simulink model "Transformer_Operating_Model_backup_before_callback_fix"  (R2025b)
settings: Solver=ode23t  StartTime=0.0  StopTime=t_stop  MaxStep=t_step_max  RelTol=1e-3
PreLoadFcn:
  | params_transformer;
InitFcn:
  | params_transformer;
undefined symbols (not defined in the file or in its folder): dT_double_age, dTheta_hr, I_LV_rated, k21, P0, P_load_min, P_tot_r, Pk, R_th_h, S_rated, theta_amb_C, theta_ref_age, x_oil, y_wdg
libraries: fl_lib x16, nesl_utility x10, ee_lib x4
settings Model: Creator=Silas Asare  LastModifiedBy=Silas Asare

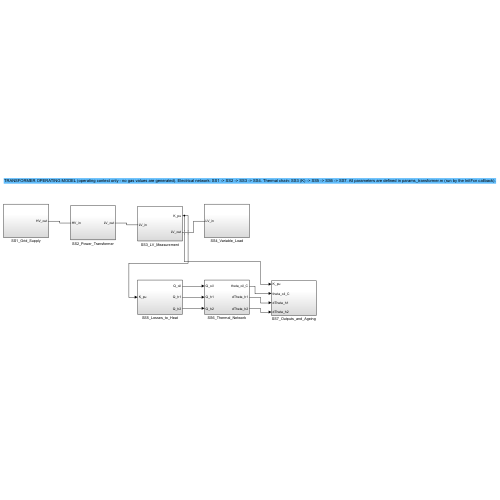
[thumbnail: Simulink's stored preview of the top-level diagram]
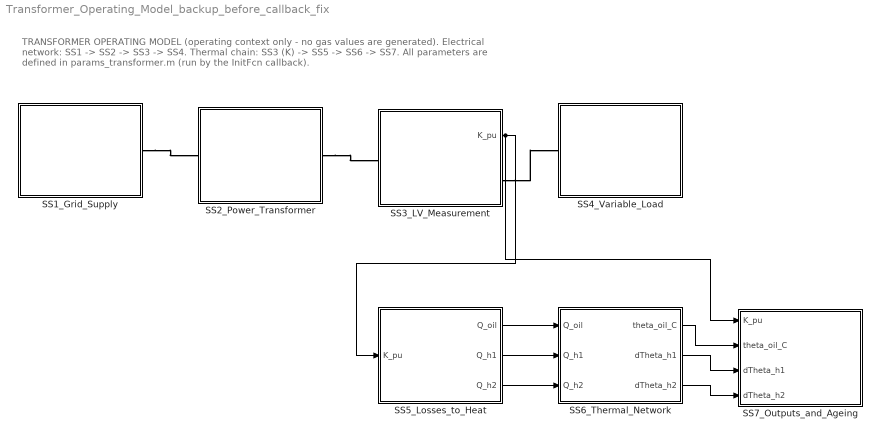
== system Transformer_Operating_Model_backup_before_callback_fix ==
  note: TRANSFORMER OPERATING MODEL (operating context only - no gas values are generated). Electrical network: SS1 -> SS2 -> SS3 -> SS4. Thermal chain: SS3 (K) -> SS5 -> SS6 -> SS7. All parameters are defined in params_transformer.m (run by the InitFcn callback).
  SS1_Grid_Supply : Subsystem
  SS2_Power_Transformer : Subsystem
  SS3_LV_Measurement : Subsystem
  SS4_Variable_Load : Subsystem
  SS5_Losses_to_Heat : Subsystem
  SS6_Thermal_Network : Subsystem
  SS7_Outputs_and_Ageing : Subsystem
  wires:
  SS3_LV_Measurement/1(K_pu) -> SS5_Losses_to_Heat/1(K_pu), SS7_Outputs_and_Ageing/1(K_pu)
  SS5_Losses_to_Heat/1(Q_oil) -> SS6_Thermal_Network/1(Q_oil)
  SS6_Thermal_Network/1(theta_oil_C) -> SS7_Outputs_and_Ageing/2(theta_oil_C)
  SS5_Losses_to_Heat/2(Q_h1) -> SS6_Thermal_Network/2(Q_h1)
  SS6_Thermal_Network/2(dTheta_h1) -> SS7_Outputs_and_Ageing/3(dTheta_h1)
  SS5_Losses_to_Heat/3(Q_h2) -> SS6_Thermal_Network/3(Q_h2)
  SS6_Thermal_Network/3(dTheta_h2) -> SS7_Outputs_and_Ageing/4(dTheta_h2)
  connections:
  SS1_Grid_Supply/RConn1 -- SS2_Power_Transformer/LConn1
  SS2_Power_Transformer/RConn1 -- SS3_LV_Measurement/LConn1
  SS3_LV_Measurement/RConn1 -- SS4_Variable_Load/LConn1

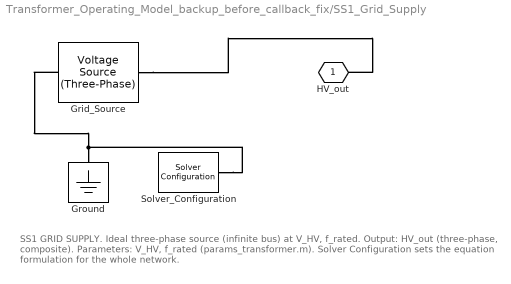
== system Transformer_Operating_Model_backup_before_callback_fix/SS1_Grid_Supply ==
  note: SS1 GRID SUPPLY. Ideal three-phase source (infinite bus) at V_HV, f_rated. Output: HV_out (three-phase, composite). Parameters: V_HV, f_rated (params_transformer.m). Solver Configuration sets the equation formulation for the whole network.
  Grid_Source : ee_lib/Sources/Voltage Source (Three-Phase)  vline_rms=V_HV V  shift=phase_shift_deg deg  freq=f_rated Hz  impedance_option=0  SShortCircuit=1e6 A*V  XR=15  R=0.01 Ohm  L=3.97e-4 H  harmonic_option=0  harmonic_orders=[5, 7, 11, 13]  harmonic_ratios=[.1, .1, .1, .1]  G_parasitic=0 1/Ohm  I_specify=off  I_priority=None  I=[0, 0, 0] A  I_nominal_specify=off  I_nominal_value=1  I_nominal_unit=A
  Ground : fl_lib/Electrical/Electrical Elements/Electrical Reference
  Solver_Configuration : nesl_utility/Solver Configuration  PhysicalDomain=network_engine_domain  SubClassName=solver  LeftPortType=input  RightPortType=generic  Tones=[]  Harmonics=[]  SimulateNoise=off  Profile=off  UseLocalSampling=off  EnableSwitchedLinearOptims=on  FrequencyDomain=off  UseCCode=off  RelTol=0.001  AbsTol=0.001  MinStep=1e-09  ToWorkspace=off  RevertToSquareIcSolve=off  NumHomotopyIterations=100  PhasorMode=off  PhasorModeNumHarmonics=1  ConsistencySolver=NEWTON_XTOL_AFTER_FTOL  IndexReductionMethod=DerivativeReplacement  DoDC=off  ResidualTolerance=1e-09  ConsistencyTolSource=GLOBAL  ConsistencyAbsTol=0.001  ConsistencyRelTol=0.001  ConsistencyTolFactor=0.001  UseLocalSolver=off  LocalSolverChoice=NE_BACKWARD_EULER_ADVANCER  ResolveIndetEquations=on  FunctionEvalNumThread=1  LocalSolverSampleTime=0.001  DoFixedCost=off  MaxNonlinIter=3  MaxModeIter=2  ComputeImpulses=off  ImpulseIterations=2  LinearAlgebra=auto  LinearAlgebraNumThread=0  EquationFormulation=NE_FREQUENCY_TIME_EF  DelaysMemoryBudget=1024  AutomaticFiltering=on  FilteringTimeConstant=0.001  PartitionStorageMethod=AS_NEEDED  PartitionMemoryBudget=1024  PartitionMethod=ROBUST  MultibodyUseLocalSolver=off  MultibodyLocalSolverChoice=ODE1  MultibodyLocalSolverSampleTime=0.001
  HV_out : PMIOPort  Side=Right
  connections:
  Ground/LConn1 -- Grid_Source/LConn1 -- Solver_Configuration/RConn1
  Grid_Source/RConn1 -- HV_out/RConn1

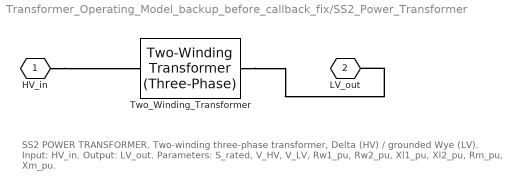
== system Transformer_Operating_Model_backup_before_callback_fix/SS2_Power_Transformer ==
  note: SS2 POWER TRANSFORMER. Two-winding three-phase transformer, Delta (HV) / grounded Wye (LV). Input: HV_in. Output: LV_out. Parameters: S_rated, V_HV, V_LV, Rw1_pu, Rw2_pu, Xl1_pu, Xl2_pu, Rm_pu, Xm_pu.
  Two_Winding_Transformer : ee_lib/Passive/Transformers/Two-Winding Transformer (Three-Phase)  SRated=S_rated V*A  FRated=f_rated Hz  Winding1Connection=ee.enum.windingconnection.delta1  VRated1=V_HV V  Winding2Connection=ee.enum.windingconnection.Yg  VRated2=V_LV V  CoreType=ee.enum.coretype.threelimb  pu_Rw1=Rw1_pu  pu_Rw2=Rw2_pu  leakage_reactance_option=ee.enum.transformer_leakage.include  pu_Xl1=Xl1_pu  pu_Xl2=Xl2_pu  magnetizing_resistance_option=ee.enum.transformer_magnetizingResistance.include  pu_Rm=Rm_pu  magnetizing_reactance_option=ee.enum.transformer_magnetizingReactance.include  saturation_option=ee.enum.transformer_saturation.exclude  pu_Xm=Xm_pu  current_data=[0, .002, 1, 2]  magnetic_flux_data=[0, 1.2, 1.5, 1.51]  pu_X0=0.5  i1_specify=off  i1_priority=None  i1=[0, 0, 0] A  i1_nominal_specify=off  i1_nominal_value=1  i1_nominal_unit=A  i2_specify=off  i2_priority=None  i2=[0, 0, 0] A  i2_nominal_specify=off  i2_nominal_value=1  i2_nominal_unit=A  phi_specify=off  phi_priority=None  phi=[0, 0, 0]  phi_nominal_specify=off  phi_nominal_value=1  phi_nominal_unit=1  power_dissipated_specify=off  power_dissipated_priority=None  power_dissipated=0 W  power_dissipated_nominal_specify=off  power_dissipated_nominal_value=1  power_dissipated_nominal_unit=W
      settings: InternalSimscapePortConfiguration="{\"Bottom\":[],\"Left\":[{\"id\":\"N1\",\"label\":\"~1\",\"type\":\"foundation.electrical.three_phase\"}],\"Right\":[{\"id\":\"N2\",\"label\":\"~2\",\"type\":\"foundation.electrical.three_phase\"}],\"Top\":[]}"
  HV_in : PMIOPort  Side=Left
  LV_out : PMIOPort  Port=2  Side=Right
  connections:
  HV_in/RConn1 -- Two_Winding_Transformer/LConn1
  Two_Winding_Transformer/RConn1 -- LV_out/RConn1

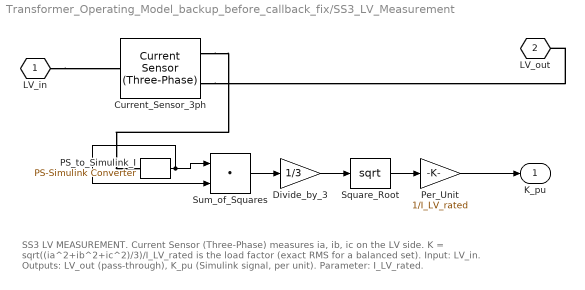
== system Transformer_Operating_Model_backup_before_callback_fix/SS3_LV_Measurement ==
  note: SS3 LV MEASUREMENT. Current Sensor (Three-Phase) measures ia, ib, ic on the LV side. K = sqrt((ia^2+ib^2+ic^2)/3)/I_LV_rated is the load factor (exact RMS for a balanced set). Input: LV_in. Outputs: LV_out (pass-through), K_pu (Simulink signal, per unit). Parameter: I_LV_rated.
  Current_Sensor_3ph : ee_lib/Sensors & Transducers/Current Sensor (Three-Phase)
  Divide_by_3 : Gain  Gain=1/3
  PS_to_Simulink_I : nesl_utility/PS-Simulink Converter  PhysicalDomain=network_engine_domain  SubClassName=ps_output  LeftPortType=input  RightPortType=output  PseudoPeriodic=off  Frequencies=[]  VectorFormat=inherit  Unit=A  AffineConversion=off
  Per_Unit : Gain  Gain=1/I_LV_rated
  Square_Root : Math  Operator=sqrt
  Sum_of_Squares : DotProduct  OutDataTypeStr=Inherit: Inherit via internal rule
  LV_in : PMIOPort  Side=Left
  LV_out : PMIOPort  Port=2  Side=Right
  K_pu : Outport
  wires:
  PS_to_Simulink_I/1 -> Sum_of_Squares/1, Sum_of_Squares/2
  Sum_of_Squares/1 -> Divide_by_3/1
  Divide_by_3/1 -> Square_Root/1
  Square_Root/1 -> Per_Unit/1
  Per_Unit/1 -> K_pu/1
  connections:
  LV_in/RConn1 -- Current_Sensor_3ph/LConn1
  Current_Sensor_3ph/RConn2 -- LV_out/RConn1
  Current_Sensor_3ph/RConn1 -- PS_to_Simulink_I/LConn1

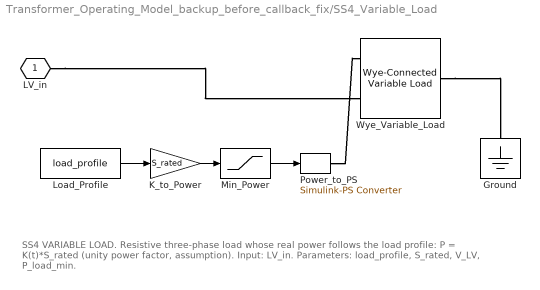
== system Transformer_Operating_Model_backup_before_callback_fix/SS4_Variable_Load ==
  note: SS4 VARIABLE LOAD. Resistive three-phase load whose real power follows the load profile: P = K(t)*S_rated (unity power factor, assumption). Input: LV_in. Parameters: load_profile, S_rated, V_LV, P_load_min.
  Ground : fl_lib/Electrical/Electrical Elements/Electrical Reference
  K_to_Power : Gain  Gain=S_rated
  Load_Profile : FromWorkspace  VariableName=load_profile  OutputAfterFinalValue=Holding final value
  Min_Power : Saturate  UpperLimit=inf  LowerLimit=P_load_min
  Power_to_PS : nesl_utility/Simulink-PS Converter  PhysicalDomain=network_engine_domain  SubClassName=ps_input  LeftPortType=input  RightPortType=output  PseudoPeriodic=off  Frequencies=[]  NoiseDistribution=none  NoiseParameters=[]  Unit=W  AffineConversion=off  FilteringAndDerivatives=provide  SimscapeFilterOrder=1  InputFilterTimeConstant=0.001  UdotUserProvided=0
  Wye_Variable_Load : ee_lib/Passive/RLC Assemblies/Wye-Connected Variable Load  VRated=V_LV V  Pmin=P_load_min W
      settings: InternalSimscapePortConfiguration="{\"Bottom\":[],\"Left\":[{\"id\":\"P\",\"label\":\"P\",\"type\":\"input\"},{\"id\":\"N\",\"label\":\"~\",\"type\":\"foundation.electrical.three_phase\"}],\"Right\":[{\"id\":\"n\",\"label\":\"n\",\"type\":\"foundation.electrical.electrical\"}],\"Top\":[]}"
  LV_in : PMIOPort  Side=Left
  wires:
  Load_Profile/1 -> K_to_Power/1
  K_to_Power/1 -> Min_Power/1
  Min_Power/1 -> Power_to_PS/1
  connections:
  LV_in/RConn1 -- Wye_Variable_Load/LConn2
  Wye_Variable_Load/RConn1 -- Ground/LConn1
  Power_to_PS/RConn1 -- Wye_Variable_Load/LConn1

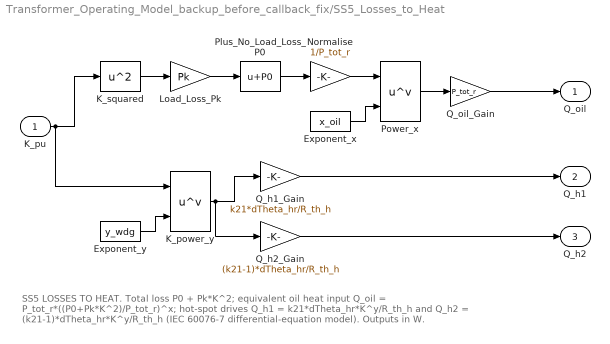
== system Transformer_Operating_Model_backup_before_callback_fix/SS5_Losses_to_Heat ==
  note: SS5 LOSSES TO HEAT. Total loss P0 + Pk*K^2; equivalent oil heat input Q_oil = P_tot_r*((P0+Pk*K^2)/P_tot_r)^x; hot-spot drives Q_h1 = k21*dTheta_hr*K^y/R_th_h and Q_h2 = (k21-1)*dTheta_hr*K^y/R_th_h (IEC 60076-7 differential-equation model). Outputs in W.
  K_pu : Inport
  Exponent_x : Constant  Value=x_oil
  Exponent_y : Constant  Value=y_wdg
  K_power_y : Math  Operator=pow
  K_squared : Math  Operator=square
  Load_Loss_Pk : Gain  Gain=Pk
  Normalise : Gain  Gain=1/P_tot_r
  Plus_No_Load_Loss_P0 : Bias  Bias=P0  SaturateOnIntegerOverflow=off
  Power_x : Math  Operator=pow
  Q_h1_Gain : Gain  Gain=k21*dTheta_hr/R_th_h
  Q_h2_Gain : Gain  Gain=(k21-1)*dTheta_hr/R_th_h
  Q_oil_Gain : Gain  Gain=P_tot_r
  Q_oil : Outport
  Q_h1 : Outport  Port=2
  Q_h2 : Outport  Port=3
  wires:
  K_pu/1 -> K_squared/1, K_power_y/1
  K_squared/1 -> Load_Loss_Pk/1
  Load_Loss_Pk/1 -> Plus_No_Load_Loss_P0/1
  Plus_No_Load_Loss_P0/1 -> Normalise/1
  Normalise/1 -> Power_x/1
  Exponent_x/1 -> Power_x/2
  Power_x/1 -> Q_oil_Gain/1
  Q_oil_Gain/1 -> Q_oil/1
  Exponent_y/1 -> K_power_y/2
  K_power_y/1 -> Q_h1_Gain/1, Q_h2_Gain/1
  Q_h1_Gain/1 -> Q_h1/1
  Q_h2_Gain/1 -> Q_h2/1

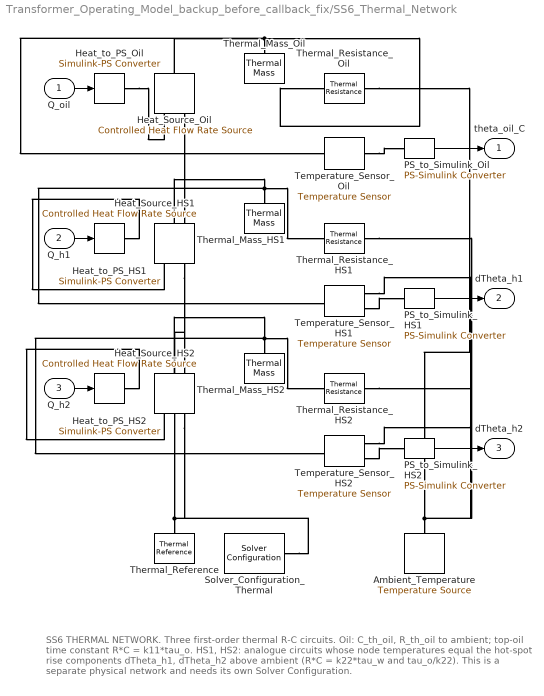
== system Transformer_Operating_Model_backup_before_callback_fix/SS6_Thermal_Network ==
  note: SS6 THERMAL NETWORK. Three first-order thermal R-C circuits. Oil: C_th_oil, R_th_oil to ambient; top-oil time constant R*C = k11*tau_o. HS1, HS2: analogue circuits whose node temperatures equal the hot-spot rise components dTheta_h1, dTheta_h2 above ambient (R*C = k22*tau_w and tau_o/k22). This is a separate physical network and needs its own Solver Configuration.
  Q_oil : Inport
  Q_h1 : Inport  Port=2
  Q_h2 : Inport  Port=3
  Ambient_Temperature : fl_lib/Thermal/Thermal Sources/Temperature Source  temperature=theta_amb_C + 273.15 K
  Heat_Source_HS1 : fl_lib/Thermal/Thermal Sources/Controlled Heat Flow Rate Source
  Heat_Source_HS2 : fl_lib/Thermal/Thermal Sources/Controlled Heat Flow Rate Source
  Heat_Source_Oil : fl_lib/Thermal/Thermal Sources/Controlled Heat Flow Rate Source
  Heat_to_PS_HS1 : nesl_utility/Simulink-PS Converter  PhysicalDomain=network_engine_domain  SubClassName=ps_input  LeftPortType=input  RightPortType=output  PseudoPeriodic=off  Frequencies=[]  NoiseDistribution=none  NoiseParameters=[]  Unit=W  AffineConversion=off  FilteringAndDerivatives=provide  SimscapeFilterOrder=1  InputFilterTimeConstant=0.001  UdotUserProvided=0
  Heat_to_PS_HS2 : nesl_utility/Simulink-PS Converter  PhysicalDomain=network_engine_domain  SubClassName=ps_input  LeftPortType=input  RightPortType=output  PseudoPeriodic=off  Frequencies=[]  NoiseDistribution=none  NoiseParameters=[]  Unit=W  AffineConversion=off  FilteringAndDerivatives=provide  SimscapeFilterOrder=1  InputFilterTimeConstant=0.001  UdotUserProvided=0
  Heat_to_PS_Oil : nesl_utility/Simulink-PS Converter  PhysicalDomain=network_engine_domain  SubClassName=ps_input  LeftPortType=input  RightPortType=output  PseudoPeriodic=off  Frequencies=[]  NoiseDistribution=none  NoiseParameters=[]  Unit=W  AffineConversion=off  FilteringAndDerivatives=provide  SimscapeFilterOrder=1  InputFilterTimeConstant=0.001  UdotUserProvided=0
  PS_to_Simulink_HS1 : nesl_utility/PS-Simulink Converter  PhysicalDomain=network_engine_domain  SubClassName=ps_output  LeftPortType=input  RightPortType=output  PseudoPeriodic=off  Frequencies=[]  VectorFormat=inherit  Unit=K  AffineConversion=off
  PS_to_Simulink_HS2 : nesl_utility/PS-Simulink Converter  PhysicalDomain=network_engine_domain  SubClassName=ps_output  LeftPortType=input  RightPortType=output  PseudoPeriodic=off  Frequencies=[]  VectorFormat=inherit  Unit=K  AffineConversion=off
  PS_to_Simulink_Oil : nesl_utility/PS-Simulink Converter  PhysicalDomain=network_engine_domain  SubClassName=ps_output  LeftPortType=input  RightPortType=output  PseudoPeriodic=off  Frequencies=[]  VectorFormat=inherit  Unit=degC  AffineConversion=on
  Solver_Configuration_Thermal : nesl_utility/Solver Configuration  PhysicalDomain=network_engine_domain  SubClassName=solver  LeftPortType=input  RightPortType=generic  Tones=[]  Harmonics=[]  SimulateNoise=off  Profile=off  UseLocalSampling=off  EnableSwitchedLinearOptims=on  FrequencyDomain=off  UseCCode=off  RelTol=0.001  AbsTol=0.001  MinStep=1e-09  ToWorkspace=off  RevertToSquareIcSolve=off  NumHomotopyIterations=100  PhasorMode=off  PhasorModeNumHarmonics=1  ConsistencySolver=NEWTON_XTOL_AFTER_FTOL  IndexReductionMethod=DerivativeReplacement  DoDC=off  ResidualTolerance=1e-09  ConsistencyTolSource=GLOBAL  ConsistencyAbsTol=0.001  ConsistencyRelTol=0.001  ConsistencyTolFactor=0.001  UseLocalSolver=off  LocalSolverChoice=NE_BACKWARD_EULER_ADVANCER  ResolveIndetEquations=on  FunctionEvalNumThread=1  LocalSolverSampleTime=0.001  DoFixedCost=off  MaxNonlinIter=3  MaxModeIter=2  ComputeImpulses=off  ImpulseIterations=2  LinearAlgebra=auto  LinearAlgebraNumThread=0  EquationFormulation=NE_TIME_EF  DelaysMemoryBudget=1024  AutomaticFiltering=on  FilteringTimeConstant=0.001  PartitionStorageMethod=AS_NEEDED  PartitionMemoryBudget=1024  PartitionMethod=ROBUST  MultibodyUseLocalSolver=off  MultibodyLocalSolverChoice=ODE1  MultibodyLocalSolverSampleTime=0.001
  Temperature_Sensor_HS1 : fl_lib/Thermal/Thermal Sensors/Temperature Sensor  temperature_measure=foundation.enum.MeasurementReference.difference
  Temperature_Sensor_HS2 : fl_lib/Thermal/Thermal Sensors/Temperature Sensor  temperature_measure=foundation.enum.MeasurementReference.difference
  Temperature_Sensor_Oil : fl_lib/Thermal/Thermal Sensors/Temperature Sensor  temperature_measure=foundation.enum.MeasurementReference.absolute
      settings: InternalSimscapePortConfiguration="{\"Bottom\":[],\"Left\":[{\"id\":\"A\",\"label\":\"A\",\"type\":\"foundation.thermal.thermal\"}],\"Right\":[{\"id\":\"T\",\"label\":\"T\",\"type\":\"output\"}],\"Top\":[]}"
  Thermal_Mass_HS1 : fl_lib/Thermal/Thermal Elements/Thermal Mass  mass_type=foundation.enum.constant_variable.constant  mass=C_th_h1 kg  sp_heat=cp_unit J/(kg*K)  mass_min=1e-6 kg  num_ports=foundation.enum.numPorts2.one  m_specify=off  m_priority=High  m=1 kg  m_nominal_specify=off  m_nominal_value=1  m_nominal_unit=kg  T_specify=on  T_priority=High  T=theta_amb_C + 273.15 K  T_nominal_specify=off  T_nominal_value=1  T_nominal_unit=K  Q_specify=off  Q_priority=None  Q=0 W  Q_nominal_specify=off  Q_nominal_value=1  Q_nominal_unit=W
  Thermal_Mass_HS2 : fl_lib/Thermal/Thermal Elements/Thermal Mass  mass_type=foundation.enum.constant_variable.constant  mass=C_th_h2 kg  sp_heat=cp_unit J/(kg*K)  mass_min=1e-6 kg  num_ports=foundation.enum.numPorts2.one  m_specify=off  m_priority=High  m=1 kg  m_nominal_specify=off  m_nominal_value=1  m_nominal_unit=kg  T_specify=on  T_priority=High  T=theta_amb_C + 273.15 K  T_nominal_specify=off  T_nominal_value=1  T_nominal_unit=K  Q_specify=off  Q_priority=None  Q=0 W  Q_nominal_specify=off  Q_nominal_value=1  Q_nominal_unit=W
  Thermal_Mass_Oil : fl_lib/Thermal/Thermal Elements/Thermal Mass  mass_type=foundation.enum.constant_variable.constant  mass=C_th_oil kg  sp_heat=cp_unit J/(kg*K)  mass_min=1e-6 kg  num_ports=foundation.enum.numPorts2.one  m_specify=off  m_priority=High  m=1 kg  m_nominal_specify=off  m_nominal_value=1  m_nominal_unit=kg  T_specify=on  T_priority=High  T=theta_amb_C + 273.15 K  T_nominal_specify=off  T_nominal_value=1  T_nominal_unit=K  Q_specify=off  Q_priority=None  Q=0 W  Q_nominal_specify=off  Q_nominal_value=1  Q_nominal_unit=W
  Thermal_Reference : fl_lib/Thermal/Thermal Elements/Thermal Reference
  Thermal_Resistance_HS1 : fl_lib/Thermal/Thermal Elements/Thermal Resistance  resistance=R_th_h K/W  T_specify=off  T_priority=None  T=0 K  T_nominal_specify=off  T_nominal_value=1  T_nominal_unit=K  Q_specify=off  Q_priority=None  Q=0 W  Q_nominal_specify=off  Q_nominal_value=1  Q_nominal_unit=W
  Thermal_Resistance_HS2 : fl_lib/Thermal/Thermal Elements/Thermal Resistance  resistance=R_th_h K/W  T_specify=off  T_priority=None  T=0 K  T_nominal_specify=off  T_nominal_value=1  T_nominal_unit=K  Q_specify=off  Q_priority=None  Q=0 W  Q_nominal_specify=off  Q_nominal_value=1  Q_nominal_unit=W
  Thermal_Resistance_Oil : fl_lib/Thermal/Thermal Elements/Thermal Resistance  resistance=R_th_oil K/W  T_specify=off  T_priority=None  T=0 K  T_nominal_specify=off  T_nominal_value=1  T_nominal_unit=K  Q_specify=off  Q_priority=None  Q=0 W  Q_nominal_specify=off  Q_nominal_value=1  Q_nominal_unit=W
  theta_oil_C : Outport
  dTheta_h1 : Outport  Port=2
  dTheta_h2 : Outport  Port=3
  wires:
  Q_oil/1 -> Heat_to_PS_Oil/1
  PS_to_Simulink_Oil/1 -> theta_oil_C/1
  Q_h1/1 -> Heat_to_PS_HS1/1
  PS_to_Simulink_HS1/1 -> dTheta_h1/1
  Q_h2/1 -> Heat_to_PS_HS2/1
  PS_to_Simulink_HS2/1 -> dTheta_h2/1
  connections:
  Heat_to_PS_Oil/RConn1 -- Heat_Source_Oil/RConn1
  Heat_Source_Oil/RConn2 -- Heat_Source_HS1/RConn2 -- Heat_Source_HS2/RConn2 -- Thermal_Reference/LConn1 -- Solver_Configuration_Thermal/RConn1
  Heat_Source_Oil/LConn1 -- Thermal_Resistance_Oil/LConn1 -- Thermal_Mass_Oil/LConn1 -- Temperature_Sensor_Oil/LConn1
  Thermal_Resistance_Oil/RConn1 -- Thermal_Resistance_HS1/RConn1 -- Temperature_Sensor_HS1/RConn1 -- Thermal_Resistance_HS2/RConn1 -- Ambient_Temperature/LConn1 -- Temperature_Sensor_HS2/RConn1
  Temperature_Sensor_Oil/RConn1 -- PS_to_Simulink_Oil/LConn1
  Heat_to_PS_HS1/RConn1 -- Heat_Source_HS1/RConn1
  Heat_Source_HS1/LConn1 -- Thermal_Resistance_HS1/LConn1 -- Thermal_Mass_HS1/LConn1 -- Temperature_Sensor_HS1/LConn1
  Temperature_Sensor_HS1/RConn2 -- PS_to_Simulink_HS1/LConn1
  Heat_to_PS_HS2/RConn1 -- Heat_Source_HS2/RConn1
  Heat_Source_HS2/LConn1 -- Thermal_Resistance_HS2/LConn1 -- Thermal_Mass_HS2/LConn1 -- Temperature_Sensor_HS2/LConn1
  Temperature_Sensor_HS2/RConn2 -- PS_to_Simulink_HS2/LConn1

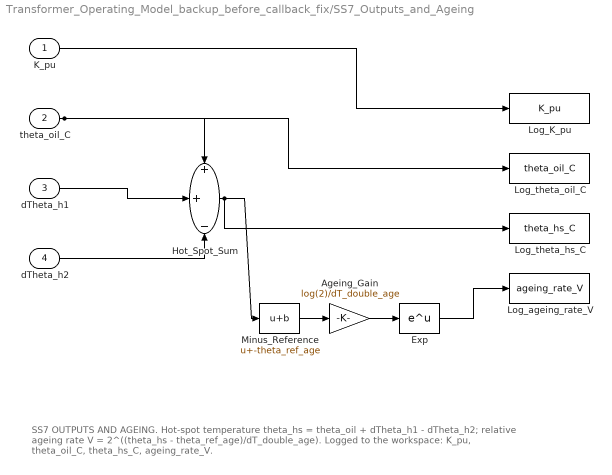
== system Transformer_Operating_Model_backup_before_callback_fix/SS7_Outputs_and_Ageing ==
  note: SS7 OUTPUTS AND AGEING. Hot-spot temperature theta_hs = theta_oil + dTheta_h1 - dTheta_h2; relative ageing rate V = 2^((theta_hs - theta_ref_age)/dT_double_age). Logged to the workspace: K_pu, theta_oil_C, theta_hs_C, ageing_rate_V.
  K_pu : Inport
  theta_oil_C : Inport  Port=2
  dTheta_h1 : Inport  Port=3
  dTheta_h2 : Inport  Port=4
  Ageing_Gain : Gain  Gain=log(2)/dT_double_age
  Exp : Math
  Hot_Spot_Sum : Sum  Inputs=++-
  Log_K_pu : ToWorkspace  VariableName=K_pu  SaveFormat=Timeseries  SampleTime=-1
  Log_ageing_rate_V : ToWorkspace  VariableName=ageing_rate_V  SaveFormat=Timeseries  SampleTime=-1
  Log_theta_hs_C : ToWorkspace  VariableName=theta_hs_C  SaveFormat=Timeseries  SampleTime=-1
  Log_theta_oil_C : ToWorkspace  VariableName=theta_oil_C  SaveFormat=Timeseries  SampleTime=-1
  Minus_Reference : Bias  Bias=-theta_ref_age  SaturateOnIntegerOverflow=off
  wires:
  theta_oil_C/1 -> Hot_Spot_Sum/1, Log_theta_oil_C/1
  dTheta_h1/1 -> Hot_Spot_Sum/2
  dTheta_h2/1 -> Hot_Spot_Sum/3
  Hot_Spot_Sum/1 -> Minus_Reference/1, Log_theta_hs_C/1
  Minus_Reference/1 -> Ageing_Gain/1
  Ageing_Gain/1 -> Exp/1
  K_pu/1 -> Log_K_pu/1
  Exp/1 -> Log_ageing_rate_V/1
